simulink subsystem "Shooting_Parameters_sub"  (R2023b)
settings: Solver=VariableStepAuto  StartTime=0.0  StopTime=10.0  RelTol=1e-3
undefined symbols (not defined in the file): Blue_Hub_LeftX, Blue_Hub_LeftY, Blue_Hub_RightX, Blue_Hub_RightY, Field_Blue_Hub_X, Field_Blue_Pass_X, Field_Hub_Y, Field_Length, Field_Length_Half, Field_Pass_Y_Bottom, Field_Pass_Y_Top, Field_Red_Hub_X, Field_Red_Pass_X, Field_Width_Pass, iterations, Rebuilt_Des_Gyro_Shoot_Offset, Rebuilt_Shoot_Dist_0, Rebuilt_Shoot_Dist_1, Rebuilt_Shoot_Dist_2, Rebuilt_Shoot_Dist_3, Rebuilt_Shoot_Dist_4, Rebuilt_Shoot_Dist_5, Rebuilt_Shoot_Dist_6, Rebuilt_Shoot_Dist_7, Rebuilt_Shoot_Gyro_Err_0, Rebuilt_Shoot_Gyro_Err_1, Rebuilt_Shoot_Gyro_Err_2, Rebuilt_Shoot_Gyro_Err_3, Rebuilt_Shoot_Gyro_Err_4, Rebuilt_Shoot_Gyro_Err_5, Rebuilt_Shoot_Gyro_Err_6, Rebuilt_Shoot_Gyro_Err_7, Rebuilt_Shoot_Hood_Pos_0, Rebuilt_Shoot_Hood_Pos_1, Rebuilt_Shoot_Hood_Pos_2, Rebuilt_Shoot_Hood_Pos_3, Rebuilt_Shoot_Hood_Pos_4, Rebuilt_Shoot_Hood_Pos_5, Rebuilt_Shoot_Hood_Pos_6, Rebuilt_Shoot_Hood_Pos_7, Rebuilt_Shoot_Shooter_Spd_0, Rebuilt_Shoot_Shooter_Spd_1, Rebuilt_Shoot_Shooter_Spd_2, Rebuilt_Shoot_Shooter_Spd_3, Rebuilt_Shoot_Shooter_Spd_4, Rebuilt_Shoot_Shooter_Spd_5, Rebuilt_Shoot_Shooter_Spd_6, Rebuilt_Shoot_Shooter_Spd_7, Rebuilt_Shoot_Shooter_Spd_I_0, Rebuilt_Shoot_Shooter_Spd_I_1, Rebuilt_Shoot_Shooter_Spd_I_2, Rebuilt_Shoot_Shooter_Spd_I_3, Rebuilt_Shoot_Shooter_Spd_I_4, Rebuilt_Shoot_Shooter_Spd_I_5, Rebuilt_Shoot_Shooter_Spd_I_6, Rebuilt_Shoot_Shooter_Spd_I_7, Rebuilt_Shoot_Target_Error_Thresh, Rebuilt_Shoot_TOF_0, Rebuilt_Shoot_TOF_1, Rebuilt_Shoot_TOF_2 ... (+11)
libraries: simulink x6, simulink_extras x2
settings Model: Creator=ander  LastModifiedBy=FIRSTMentor

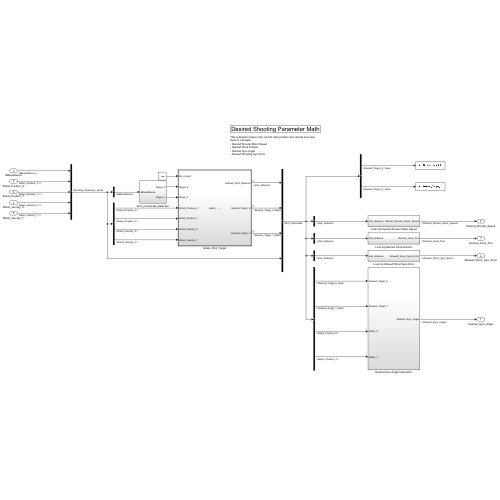
[thumbnail: Simulink's stored preview of the top-level diagram]
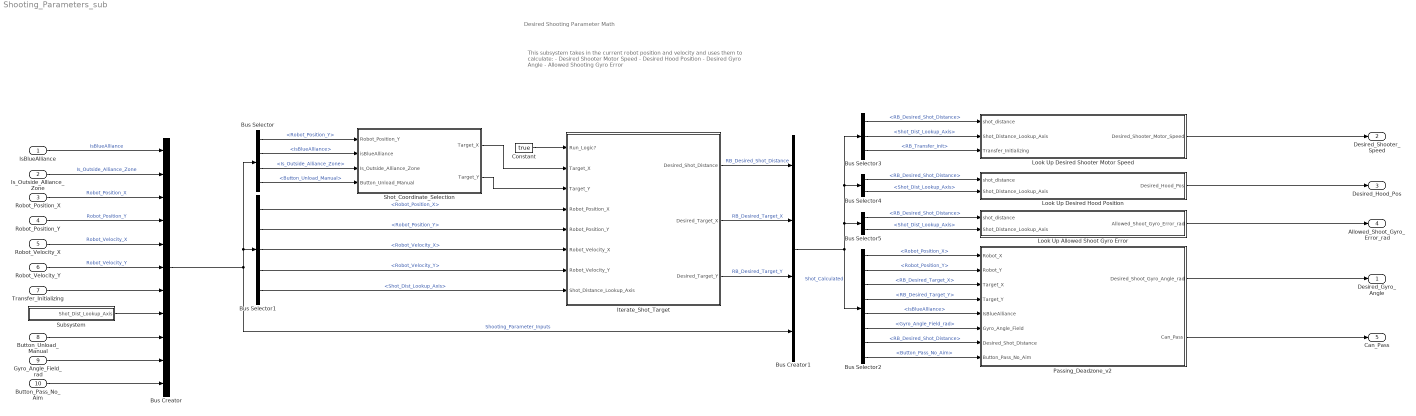
== system Shooting_Parameters_sub ==
  note: Desired Shooting Parameter Math
  note: This subsystem takes in the current robot position and velocity and uses them to calculate:
      | - Desired Shooter Motor Speed
      | - Desired Hood Position
      | - Desired Gyro Angle
      | - Allowed Shooting Gyro Error
  IsBlueAlliance : Inport
  Is_Outside_Alliance_Zone : Inport  Port=2
  Robot_Position_X : Inport  Port=3
  Robot_Position_Y : Inport  Port=4
  Robot_Velocity_X : Inport  Port=5
  Robot_Velocity_Y : Inport  Port=6
  Transfer_Initializing : Inport  Port=7
  Button_Unload_Manual : Inport  Port=8
  Gyro_Angle_Field_rad : Inport  Port=9
  Button_Pass_No_Aim : Inport  Port=10
  Bus Creator : BusCreator  Inputs=11
  Bus Creator1 : BusCreator  Inputs=4
  Bus Selector : BusSelector  OutputSignals=Robot_Position_Y,IsBlueAlliance,Is_Outside_Alliance_Zone,Button_Unload_Manual
  Bus Selector1 : BusSelector  OutputSignals=Robot_Position_X,Robot_Position_Y,Robot_Velocity_X,Robot_Velocity_Y,Shot_Dist_Lookup_Axis
  Bus Selector2 : BusSelector  OutputSignals=Shooting_Parameter_Inputs.Robot_Position_X,Shooting_Parameter_Inputs.Robot_Position_Y,RB_Desired_Target_X,RB_Desired_Target_Y,Shooting_Parameter_Inputs.IsBlueAlliance,Shooting_Parameter_Inputs.Gyro_Angle_Field_rad,RB_Desired_Shot_Distance,Shooting_Parameter_Inputs.Button_Pass_No_Aim
  Bus Selector3 : BusSelector  OutputSignals=RB_Desired_Shot_Distance,Shooting_Parameter_Inputs.Shot_Dist_Lookup_Axis,Shooting_Parameter_Inputs.RB_Transfer_Init
  Bus Selector4 : BusSelector  OutputSignals=RB_Desired_Shot_Distance,Shooting_Parameter_Inputs.Shot_Dist_Lookup_Axis
  Bus Selector5 : BusSelector  OutputSignals=RB_Desired_Shot_Distance,Shooting_Parameter_Inputs.Shot_Dist_Lookup_Axis
  Constant : Constant  Value=true  OutDataTypeStr=boolean
  Iterate_Shot_Target : Subsystem  TreatAsAtomicUnit=on
  Look Up Allowed Shoot Gyro Error : Subsystem
  Look Up Desired Hood Position : Subsystem
  Look Up Desired Shooter Motor Speed : Subsystem
  Passing_Deadzone_v2 : Subsystem
  Shot_Coordinate_Selection : Subsystem
  Subsystem : Subsystem
  Desired_Gyro_Angle : Outport
  Desired_Shooter_Speed : Outport  Port=2
  Desired_Hood_Pos : Outport  Port=3
  Allowed_Shoot_Gyro_Error_rad : Outport  Port=4
  Can_Pass : Outport  Port=5
  wires:
  Robot_Position_X/1 -> Bus Creator/3  "Robot_Position_X"
  Constant/1 -> Iterate_Shot_Target/1(Run_Logic?)
  Bus Selector1/2 -> Iterate_Shot_Target/5(Robot_Position_Y)  "<Robot_Position_Y>"
  Look Up Desired Hood Position/1(Desired_Hood_Pos) -> Desired_Hood_Pos/1
  Robot_Position_Y/1 -> Bus Creator/4  "Robot_Position_Y"
  Bus Selector/2 -> Shot_Coordinate_Selection/2(isBlueAlliance)  "<IsBlueAlliance>"
  Iterate_Shot_Target/2(Desired_Target_X) -> Bus Creator1/2  "RB_Desired_Target_X"
  Bus Selector4/1 -> Look Up Desired Hood Position/1(shot_distance)  "<RB_Desired_Shot_Distance>"
  Shot_Coordinate_Selection/1(Target_X) -> Iterate_Shot_Target/2(Target_X)
  Bus Creator/1 -> Bus Creator1/4, Bus Selector1/1, Bus Selector/1  "Shooting_Parameter_Inputs"
  Look Up Desired Shooter Motor Speed/1(Desired_Shooter_Motor_Speed) -> Desired_Shooter_Speed/1
  Bus Creator1/1 -> Bus Selector2/1, Bus Selector5/1, Bus Selector3/1, Bus Selector4/1  "Shot_Calculated"
  Shot_Coordinate_Selection/2(Target_Y) -> Iterate_Shot_Target/3(Target_Y)
  Bus Selector3/1 -> Look Up Desired Shooter Motor Speed/1(shot_distance)  "<RB_Desired_Shot_Distance>"
  Robot_Velocity_X/1 -> Bus Creator/5  "Robot_Velocity_X"
  Bus Selector5/1 -> Look Up Allowed Shoot Gyro Error/1(shot_distance)  "<RB_Desired_Shot_Distance>"
  Iterate_Shot_Target/1(Desired_Shot_Distance) -> Bus Creator1/1  "RB_Desired_Shot_Distance"
  Bus Selector1/4 -> Iterate_Shot_Target/7(Robot_Velocity_Y)  "<Robot_Velocity_Y>"
  Bus Selector1/1 -> Iterate_Shot_Target/4(Robot_Position_X)  "<Robot_Position_X>"
  Bus Selector1/3 -> Iterate_Shot_Target/6(Robot_Velocity_X)  "<Robot_Velocity_X>"
  Robot_Velocity_Y/1 -> Bus Creator/6  "Robot_Velocity_Y"
  Look Up Allowed Shoot Gyro Error/1(Allowed_Shoot_Gyro_Error_rad) -> Allowed_Shoot_Gyro_Error_rad/1
  Iterate_Shot_Target/3(Desired_Target_Y) -> Bus Creator1/3  "RB_Desired_Target_Y"
  Subsystem/1(Shot_Dist_Lookup_Axis) -> Bus Creator/8
  Bus Selector3/2 -> Look Up Desired Shooter Motor Speed/2(Shot_Distance_Lookup_Axis)  "<Shot_Dist_Lookup_Axis>"
  Bus Selector5/2 -> Look Up Allowed Shoot Gyro Error/2(Shot_Distance_Lookup_Axis)  "<Shot_Dist_Lookup_Axis>"
  Bus Selector4/2 -> Look Up Desired Hood Position/2(Shot_Distance_Lookup_Axis)  "<Shot_Dist_Lookup_Axis>"
  Bus Selector1/5 -> Iterate_Shot_Target/8(Shot_Distance_Lookup_Axis)  "<Shot_Dist_Lookup_Axis>"
  Bus Selector/1 -> Shot_Coordinate_Selection/1(Robot_Position_Y)  "<Robot_Position_Y>"
  Bus Selector/3 -> Shot_Coordinate_Selection/3(Is_Outside_Alliance_Zone)  "<Is_Outside_Alliance_Zone>"
  IsBlueAlliance/1 -> Bus Creator/1  "IsBlueAlliance"
  Is_Outside_Alliance_Zone/1 -> Bus Creator/2  "Is_Outside_Alliance_Zone"
  Transfer_Initializing/1 -> Bus Creator/7
  Bus Selector3/3 -> Look Up Desired Shooter Motor Speed/3(Transfer_Initializing)  "<RB_Transfer_Init>"
  Button_Unload_Manual/1 -> Bus Creator/9
  Bus Selector/4 -> Shot_Coordinate_Selection/4(Button_Unload_Manual)  "<Button_Unload_Manual>"
  Gyro_Angle_Field_rad/1 -> Bus Creator/10
  Button_Pass_No_Aim/1 -> Bus Creator/11
  Bus Selector2/1 -> Passing_Deadzone_v2/1(Robot_X)  "<Robot_Position_X>"
  Bus Selector2/2 -> Passing_Deadzone_v2/2(Robot_Y)  "<Robot_Position_Y>"
  Bus Selector2/3 -> Passing_Deadzone_v2/3(Target_X)  "<RB_Desired_Target_X>"
  Bus Selector2/4 -> Passing_Deadzone_v2/4(Target_Y)  "<RB_Desired_Target_Y>"
  Bus Selector2/5 -> Passing_Deadzone_v2/5(IsBlueAlliance)  "<IsBlueAlliance>"
  Bus Selector2/6 -> Passing_Deadzone_v2/6(Gyro_Angle_Field)  "<Gyro_Angle_Field_rad>"
  Bus Selector2/7 -> Passing_Deadzone_v2/7(Desired_Shot_Distance)  "<RB_Desired_Shot_Distance>"
  Bus Selector2/8 -> Passing_Deadzone_v2/8(Button_Pass_No_Aim)  "<Button_Pass_No_Aim>"
  Passing_Deadzone_v2/1(Desired_Shoot_Gyro_Angle_rad) -> Desired_Gyro_Angle/1
  Passing_Deadzone_v2/2(Can_Pass) -> Can_Pass/1

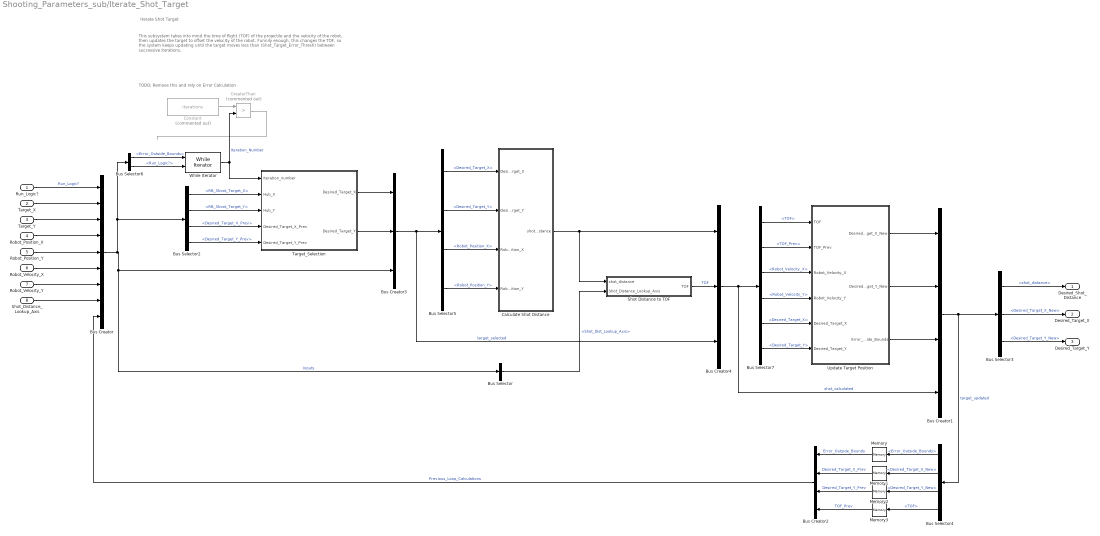
== system Shooting_Parameters_sub/Iterate_Shot_Target ==
  note: Iterate Shot Target
  note: This subsystem takes into mind the time of flight (TOF) of the projectile and the velocity of the robot, then updates the target to offset the velocity of the robot. Funnily enough, this changes the TOF, so the system keeps updating until the target moves less than (Shot_Target_Error_Thresh) between successive iterations.
  note: TODO: Remove this and rely on Error Calculation
  Run_Logic? : Inport
  Target_X : Inport  Port=2
  Target_Y : Inport  Port=3
  Robot_Position_X : Inport  Port=4
  Robot_Position_Y : Inport  Port=5
  Robot_Velocity_X : Inport  Port=6
  Robot_Velocity_Y : Inport  Port=7
  Shot_Distance_Lookup_Axis : Inport  Port=8
  Bus Creator : BusCreator  Inputs=9
  Bus Creator1 : BusCreator  Inputs=4
  Bus Creator2 : BusCreator  Inputs=4
  Bus Creator3 : BusCreator  Inputs=3
  Bus Creator4 : BusCreator  Inputs=3
  Bus Selector : BusSelector  OutputSignals=Shot_Dist_Lookup_Axis
  Bus Selector2 : BusSelector  OutputSignals=RB_Shoot_Target_X,RB_Shoot_Target_Y,Previous_Loop_Calculations.Desired_Target_X_Prev,Previous_Loop_Calculations.Desired_Target_Y_Prev
  Bus Selector3 : BusSelector  OutputSignals=shot_calculated.shot_distance,Desired_Target_X_New,Desired_Target_Y_New
  Bus Selector4 : BusSelector  OutputSignals=Error_Outside_Bounds,Desired_Target_X_New,Desired_Target_Y_New,shot_calculated.TOF
  Bus Selector5 : BusSelector  OutputSignals=Desired_Target_X,Desired_Target_Y,Inputs.Robot_Position_X,Inputs.Robot_Position_Y
  Bus Selector6 : BusSelector  OutputSignals=Previous_Loop_Calculations.Error_Outside_Bounds,Run_Logic?
  Bus Selector7 : BusSelector  OutputSignals=TOF,target_selected.Inputs.Previous_Loop_Calculations.TOF_Prev,target_selected.Inputs.Robot_Velocity_X,target_selected.Inputs.Robot_Velocity_Y,target_selected.Desired_Target_X,target_selected.Desired_Target_Y
  Calculate Shot Distance : Subsystem
  Constant : Constant  Commented=on  Value=iterations
  GreaterThan : RelationalOperator  Commented=on  Operator=>  OutDataTypeStr=boolean  RndMeth=Simplest  InputSameDT=off
  Memory : Memory  InitialCondition=true  InheritSampleTime=on
  Memory1 : Memory  InheritSampleTime=on
  Memory2 : Memory  InheritSampleTime=on
  Memory3 : Memory  InheritSampleTime=on
  Shot Distance to TOF : Subsystem
  Target_Selection : Subsystem
  Update Target Position : Subsystem
  While Iterator : WhileIterator  MaxIters=10  ResetStates=reset  ShowIterationPort=on  OutputDataType=uint8
  Desired_Shot_Distance : Outport
  Desired_Target_X : Outport  Port=2
  Desired_Target_Y : Outport  Port=3
  wires:
  Bus Selector/1 -> Shot Distance to TOF/2(Shot_Distance_Lookup_Axis)  "<Shot_Dist_Lookup_Axis>"
  Shot_Distance_Lookup_Axis/1 -> Bus Creator/8
  Robot_Velocity_Y/1 -> Bus Creator/7
  Robot_Velocity_X/1 -> Bus Creator/6
  Robot_Position_Y/1 -> Bus Creator/5
  GreaterThan/1 -> ?
  Constant/1 -> GreaterThan/1
  Bus Selector7/2 -> Update Target Position/2(TOF_Prev)  "<TOF_Prev>"
  Bus Selector3/1 -> Desired_Shot_Distance/1  "<shot_distance>"
  Bus Selector7/6 -> Update Target Position/6(Desired_Target_Y)  "<Desired_Target_Y>"
  Bus Selector7/5 -> Update Target Position/5(Desired_Target_X)  "<Desired_Target_X>"
  Bus Selector7/4 -> Update Target Position/4(Robot_Velocity_Y)  "<Robot_Velocity_Y>"
  Bus Selector7/3 -> Update Target Position/3(Robot_Velocity_X)  "<Robot_Velocity_X>"
  Bus Selector7/1 -> Update Target Position/1(TOF)  "<TOF>"
  Bus Creator4/1 -> Bus Creator1/4, Bus Selector7/1  "shot_calculated"
  Bus Selector4/4 -> Memory3/1  "<TOF>"
  Memory3/1 -> Bus Creator2/4  "TOF_Prev"
  Bus Selector5/4 -> Calculate Shot Distance/4(Robot_Position_Y)  "<Robot_Position_Y>"
  Bus Selector5/3 -> Calculate Shot Distance/3(Robot_Position_X)  "<Robot_Position_X>"
  Bus Selector5/2 -> Calculate Shot Distance/2(Desired_Target_Y)  "<Desired_Target_Y>"
  Bus Selector5/1 -> Calculate Shot Distance/1(Desired_Target_X)  "<Desired_Target_X>"
  Bus Creator3/1 -> Bus Selector5/1, Bus Creator4/3  "target_selected"
  Target_Selection/2(Desired_Target_Y) -> Bus Creator3/2
  Target_Selection/1(Desired_Target_X) -> Bus Creator3/1
  Bus Selector2/4 -> Target_Selection/5(Desired_Target_Y_Prev)  "<Desired_Target_Y_Prev>"
  Bus Selector2/3 -> Target_Selection/4(Desired_Target_X_Prev)  "<Desired_Target_X_Prev>"
  Bus Selector6/2 -> While Iterator/2  "<Run_Logic?>"
  Bus Selector6/1 -> While Iterator/1  "<Error_Outside_Bounds>"
  Bus Creator2/1 -> Bus Creator/9  "Previous_Loop_Calculations"
  Memory/1 -> Bus Creator2/1  "Error_Outside_Bounds"
  Memory2/1 -> Bus Creator2/3  "Desired_Target_Y_Prev"
  Memory1/1 -> Bus Creator2/2  "Desired_Target_X_Prev"
  Bus Selector4/3 -> Memory2/1  "<Desired_Target_Y_New>"
  Bus Selector4/2 -> Memory1/1  "<Desired_Target_X_New>"
  Bus Selector4/1 -> Memory/1  "<Error_Outside_Bounds>"
  Update Target Position/3(Error_Outside_Bounds) -> Bus Creator1/3
  Bus Selector3/3 -> Desired_Target_Y/1  "<Desired_Target_Y_New>"
  Bus Creator1/1 -> Bus Selector4/1, Bus Selector3/1  "target_updated"
  Bus Selector3/2 -> Desired_Target_X/1  "<Desired_Target_X_New>"
  Bus Selector2/2 -> Target_Selection/3(Hub_Y)  "<RB_Shoot_Target_Y>"
  Bus Selector2/1 -> Target_Selection/2(Hub_X)  "<RB_Shoot_Target_X>"
  Update Target Position/2(Desired_Target_Y_New) -> Bus Creator1/2
  Update Target Position/1(Desired_Target_X_New) -> Bus Creator1/1
  Bus Creator/1 -> Bus Selector2/1, Bus Selector6/1, Bus Creator3/3, Bus Selector/1  "Inputs"
  Target_X/1 -> Bus Creator/2
  Robot_Position_X/1 -> Bus Creator/4
  Target_Y/1 -> Bus Creator/3
  Shot Distance to TOF/1(TOF) -> Bus Creator4/2  "TOF"
  Calculate Shot Distance/1(shot_distance) -> Bus Creator4/1, Shot Distance to TOF/1(shot_distance)
  While Iterator/1 -> Target_Selection/1(iteration_number), GreaterThan/2  "Iteration_Number"
  Run_Logic?/1 -> Bus Creator/1  "Run_Logic?"

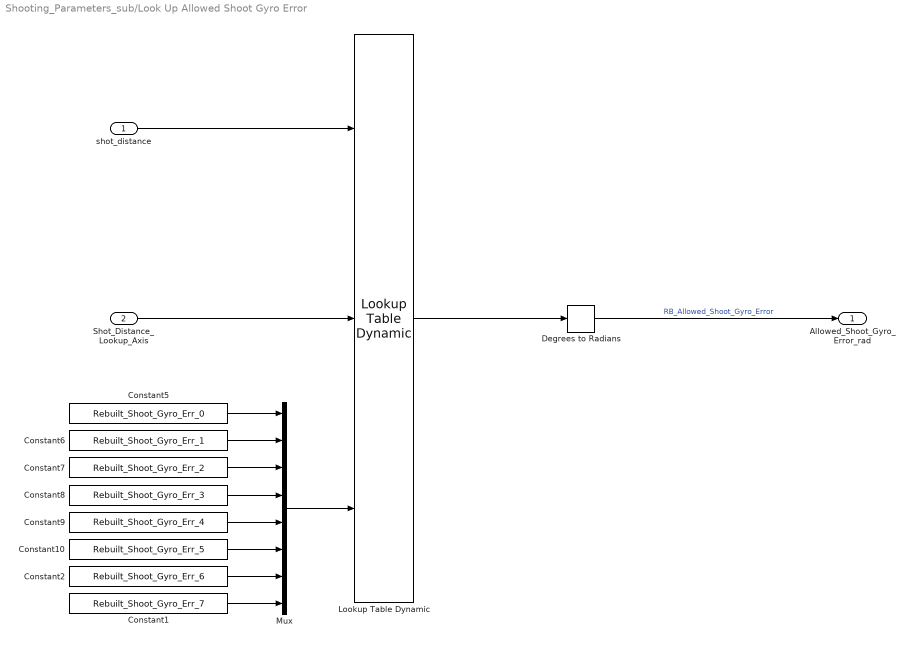
== system Shooting_Parameters_sub/Look Up Allowed Shoot Gyro Error ==
  shot_distance : Inport
  Shot_Distance_Lookup_Axis : Inport  Port=2
  Constant1 : Constant  Value=Rebuilt_Shoot_Gyro_Err_7
  Constant10 : Constant  Value=Rebuilt_Shoot_Gyro_Err_5
  Constant2 : Constant  Value=Rebuilt_Shoot_Gyro_Err_6
  Constant5 : Constant  Value=Rebuilt_Shoot_Gyro_Err_0
  Constant6 : Constant  Value=Rebuilt_Shoot_Gyro_Err_1
  Constant7 : Constant  Value=Rebuilt_Shoot_Gyro_Err_2
  Constant8 : Constant  Value=Rebuilt_Shoot_Gyro_Err_3
  Constant9 : Constant  Value=Rebuilt_Shoot_Gyro_Err_4
  Degrees to Radians : simulink_extras/Transformations/Degrees to Radians
  Lookup Table Dynamic : simulink/Lookup Tables/Lookup Table Dynamic  LookUpMeth=Interpolation-Use End Values  OutDataType=fixdt('double')  OutScaling=[]  OutputDataTypeScalingMode=Specify via dialog  OutDataTypeStr=double  DoSatur=off
  Mux : Mux  Inputs=8
  Allowed_Shoot_Gyro_Error_rad : Outport
  wires:
  Constant6/1 -> Mux/2
  Constant10/1 -> Mux/6
  Constant9/1 -> Mux/5
  Constant1/1 -> Mux/8
  Constant5/1 -> Mux/1
  Constant2/1 -> Mux/7
  Constant7/1 -> Mux/3
  Constant8/1 -> Mux/4
  Mux/1 -> Lookup Table Dynamic/3
  Shot_Distance_Lookup_Axis/1 -> Lookup Table Dynamic/2
  Degrees to Radians/1 -> Allowed_Shoot_Gyro_Error_rad/1  "RB_Allowed_Shoot_Gyro_Error"
  Lookup Table Dynamic/1 -> Degrees to Radians/1
  shot_distance/1 -> Lookup Table Dynamic/1

== system Shooting_Parameters_sub/Look Up Desired Hood Position ==
  shot_distance : Inport
  Shot_Distance_Lookup_Axis : Inport  Port=2
  Constant1 : Constant  Value=Rebuilt_Shoot_Hood_Pos_7
  Constant10 : Constant  Value=Rebuilt_Shoot_Hood_Pos_5
  Constant2 : Constant  Value=Rebuilt_Shoot_Hood_Pos_6
  Constant5 : Constant  Value=Rebuilt_Shoot_Hood_Pos_0
  Constant6 : Constant  Value=Rebuilt_Shoot_Hood_Pos_1
  Constant7 : Constant  Value=Rebuilt_Shoot_Hood_Pos_2
  Constant8 : Constant  Value=Rebuilt_Shoot_Hood_Pos_3
  Constant9 : Constant  Value=Rebuilt_Shoot_Hood_Pos_4
  Lookup Table Dynamic : simulink/Lookup Tables/Lookup Table Dynamic  LookUpMeth=Interpolation-Use End Values  OutDataType=fixdt('double')  OutScaling=[]  OutputDataTypeScalingMode=Specify via dialog  OutDataTypeStr=double  DoSatur=off
  Mux : Mux  Inputs=8
  Desired_Hood_Pos : Outport
  wires:
  Mux/1 -> Lookup Table Dynamic/3
  Constant2/1 -> Mux/7
  Constant6/1 -> Mux/2
  Constant10/1 -> Mux/6
  Constant1/1 -> Mux/8
  Constant5/1 -> Mux/1
  Constant9/1 -> Mux/5
  Constant7/1 -> Mux/3
  Constant8/1 -> Mux/4
  Shot_Distance_Lookup_Axis/1 -> Lookup Table Dynamic/2
  Lookup Table Dynamic/1 -> Desired_Hood_Pos/1
  shot_distance/1 -> Lookup Table Dynamic/1

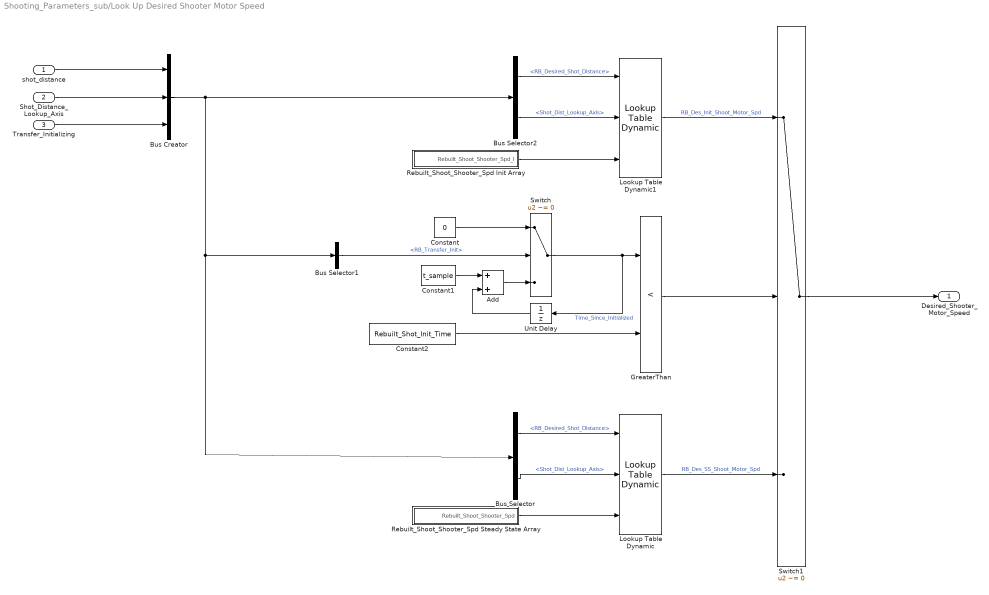
== system Shooting_Parameters_sub/Look Up Desired Shooter Motor Speed ==
  shot_distance : Inport
  Shot_Distance_Lookup_Axis : Inport  Port=2
  Transfer_Initializing : Inport  Port=3
  Add : Sum
  Bus Creator : BusCreator  Inputs=3
  Bus Selector : BusSelector  OutputSignals=RB_Desired_Shot_Distance,Shot_Dist_Lookup_Axis
  Bus Selector1 : BusSelector  OutputSignals=RB_Transfer_Init
  Bus Selector2 : BusSelector  OutputSignals=RB_Desired_Shot_Distance,Shot_Dist_Lookup_Axis
  Constant : Constant  Value=0
  Constant1 : Constant  Value=t_sample
  Constant2 : Constant  Value=Rebuilt_Shot_Init_Time
  GreaterThan : RelationalOperator  Operator=<  OutDataTypeStr=boolean  RndMeth=Simplest  InputSameDT=off
  Lookup Table Dynamic : simulink/Lookup Tables/Lookup Table Dynamic  LookUpMeth=Interpolation-Use End Values  OutDataType=fixdt('double')  OutScaling=[]  OutputDataTypeScalingMode=Specify via dialog  OutDataTypeStr=double  DoSatur=off
  Lookup Table Dynamic1 : simulink/Lookup Tables/Lookup Table Dynamic  LookUpMeth=Interpolation-Use End Values  OutDataType=fixdt('double')  OutScaling=[]  OutputDataTypeScalingMode=Specify via dialog  OutDataTypeStr=double  DoSatur=off
  Rebuilt_Shoot_Shooter_Spd Init Array : Subsystem
  Rebuilt_Shoot_Shooter_Spd Steady State Array : Subsystem
  Switch : Switch  Criteria=u2 ~= 0  SaturateOnIntegerOverflow=off  InputSameDT=off
  Switch1 : Switch  Criteria=u2 ~= 0  SaturateOnIntegerOverflow=off  InputSameDT=off
  Unit Delay : UnitDelay  SampleTime=-1  HasFrameUpgradeWarning=on
  Desired_Shooter_Motor_Speed : Outport
  wires:
  GreaterThan/1 -> Switch1/2
  Lookup Table Dynamic/1 -> Switch1/3  "RB_Des_SS_Shoot_Motor_Spd"
  Lookup Table Dynamic1/1 -> Switch1/1  "RB_Des_Init_Shoot_Motor_Spd"
  Rebuilt_Shoot_Shooter_Spd Init Array/1(Rebuilt_Shoot_Shooter_Spd_I) -> Lookup Table Dynamic1/3
  Bus Selector2/1 -> Lookup Table Dynamic1/1  "<RB_Desired_Shot_Distance>"
  Bus Selector2/2 -> Lookup Table Dynamic1/2  "<Shot_Dist_Lookup_Axis>"
  Bus Creator/1 -> Bus Selector1/1, Bus Selector/1, Bus Selector2/1
  Constant2/1 -> GreaterThan/2
  Add/1 -> Switch/3
  Constant1/1 -> Add/1
  Unit Delay/1 -> Add/2
  Constant/1 -> Switch/1
  Switch/1 -> GreaterThan/1, Unit Delay/1  "Time_Since_Initialized"
  Bus Selector1/1 -> Switch/2  "<RB_Transfer_Init>"
  Rebuilt_Shoot_Shooter_Spd Steady State Array/1(Rebuilt_Shoot_Shooter_Spd) -> Lookup Table Dynamic/3
  Bus Selector/2 -> Lookup Table Dynamic/2  "<Shot_Dist_Lookup_Axis>"
  Bus Selector/1 -> Lookup Table Dynamic/1  "<RB_Desired_Shot_Distance>"
  Transfer_Initializing/1 -> Bus Creator/3
  Shot_Distance_Lookup_Axis/1 -> Bus Creator/2
  Switch1/1 -> Desired_Shooter_Motor_Speed/1
  shot_distance/1 -> Bus Creator/1

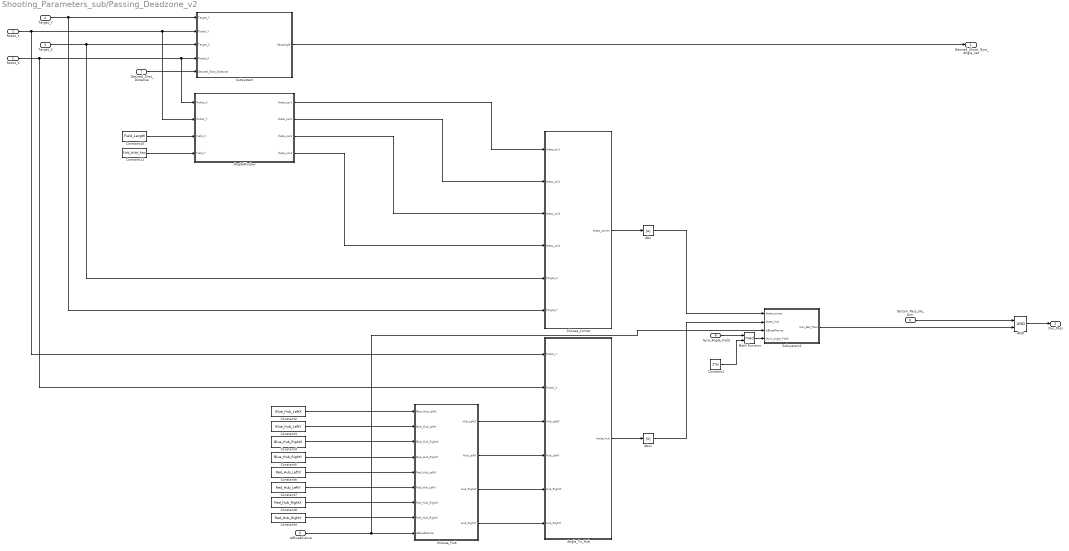
== system Shooting_Parameters_sub/Passing_Deadzone_v2 ==
  Robot_X : Inport
  Robot_Y : Inport  Port=2
  Target_X : Inport  Port=3
  Target_Y : Inport  Port=4
  IsBlueAlliance : Inport  Port=5
  Gyro_Angle_Field : Inport  Port=6
  Desired_Shot_Distance : Inport  Port=7
  Button_Pass_No_Aim : Inport  Port=8
  AND : Logic  AllPortsSameDT=off  OutDataTypeStr=boolean
  Abs : Abs  SaturateOnIntegerOverflow=off
  Abs1 : Abs  SaturateOnIntegerOverflow=off
  AngleWindow : Subsystem
  Angle_To_Hub : Subsystem
  Choose_Corner : Subsystem
  Choose_Hub : Subsystem
  Constant1 : Constant  Value=2*pi
  Constant10 : Constant  Value=Field_Length
  Constant11 : Constant  Value=Field_Width_Pass
  Constant2 : Constant  Value=Blue_Hub_LeftX
  Constant3 : Constant  Value=Blue_Hub_LeftY
  Constant4 : Constant  Value=Blue_Hub_RightX
  Constant5 : Constant  Value=Blue_Hub_RightY
  Constant6 : Constant  Value=Red_Hub_LeftX
  Constant7 : Constant  Value=Red_Hub_LeftY
  Constant8 : Constant  Value=Red_Hub_RightX
  Constant9 : Constant  Value=Red_Hub_RightY
  Math Function : Math  Operator=mod
  Subsystem : Subsystem
  Subsystem1 : Subsystem
  Desired_Shoot_Gyro_Angle_rad : Outport
  Can_Pass : Outport  Port=2
  wires:
  Button_Pass_No_Aim/1 -> AND/1
  Math Function/1 -> Subsystem1/4(Gyro_Angle_Field)
  Gyro_Angle_Field/1 -> Math Function/1
  Constant1/1 -> Math Function/2
  Subsystem1/1(Can_Bot_Pass) -> AND/2
  Abs1/1 -> Subsystem1/2(theta_hub)
  Abs/1 -> Subsystem1/1(theta_corner)
  AND/1 -> Can_Pass/1
  Desired_Shot_Distance/1 -> Subsystem/5(Desired_Shot_Distance)
  Constant11/1 -> AngleWindow/4(Field_Y)
  Constant3/1 -> Choose_Hub/2(Blue_Hub_LeftY)
  Subsystem/1(PassAngle) -> Desired_Shoot_Gyro_Angle_rad/1
  Angle_To_Hub/1(theta_hub) -> Abs1/1
  Choose_Corner/1(theta_corner) -> Abs/1
  Choose_Hub/4(Hub_RightY) -> Angle_To_Hub/6(Hub_RightY)
  Choose_Hub/3(Hub_RightX) -> Angle_To_Hub/5(Hub_RightX)
  Choose_Hub/2(Hub_LeftY) -> Angle_To_Hub/4(Hub_LeftY)
  Choose_Hub/1(Hub_LeftX) -> Angle_To_Hub/3(Hub_LeftX)
  IsBlueAlliance/1 -> Choose_Hub/9(IsBlueAlliance), Subsystem1/3(IsBlueAlliance)
  Constant9/1 -> Choose_Hub/8(Red_Hub_RightY)
  Constant8/1 -> Choose_Hub/7(Red_Hub_RightX)
  Constant7/1 -> Choose_Hub/6(Red_Hub_LeftY)
  Constant6/1 -> Choose_Hub/5(Red_Hub_LeftX)
  Constant5/1 -> Choose_Hub/4(Blue_Hub_RightY)
  Constant4/1 -> Choose_Hub/3(Blue_Hub_RightX)
  Constant2/1 -> Choose_Hub/1(Blue_Hub_LeftX)
  AngleWindow/4(theta_cor4) -> Choose_Corner/4(theta_cor4)
  AngleWindow/3(theta_cor3) -> Choose_Corner/3(theta_cor3)
  AngleWindow/2(theta_cor2) -> Choose_Corner/2(theta_cor2)
  AngleWindow/1(theta_cor1) -> Choose_Corner/1(theta_cor1)
  Constant10/1 -> AngleWindow/3(Field_X)
  Robot_X/1 -> Angle_To_Hub/2(Robot_X), Subsystem/4(Robot_X), AngleWindow/1(Robot_X)
  Target_X/1 -> Subsystem/3(Target_X), Choose_Corner/5(Target_X)
  Robot_Y/1 -> Subsystem/2(Robot_Y), AngleWindow/2(Robot_Y), Angle_To_Hub/1(Robot_Y)
  Target_Y/1 -> Subsystem/1(Target_Y), Choose_Corner/6(Target_Y)

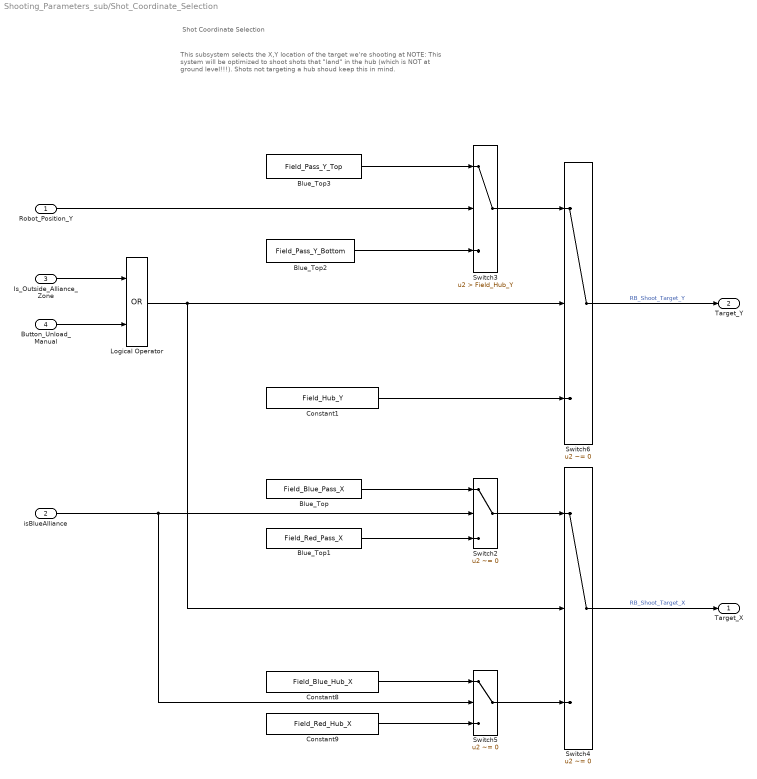
== system Shooting_Parameters_sub/Shot_Coordinate_Selection ==
  note: Shot Coordinate Selection
  note: This subsystem selects the X,Y location of the target we're shooting at
      |
      | NOTE: This system will be optimized to shoot shots that "land" in the hub (which is NOT at ground level!!!). Shots not targeting a hub shoud keep this in mind.
  Robot_Position_Y : Inport
  isBlueAlliance : Inport  Port=2
  Is_Outside_Alliance_Zone : Inport  Port=3
  Button_Unload_Manual : Inport  Port=4
  Blue_Top : Constant  Value=Field_Blue_Pass_X
  Blue_Top1 : Constant  Value=Field_Red_Pass_X
  Blue_Top2 : Constant  Value=Field_Pass_Y_Bottom
  Blue_Top3 : Constant  Value=Field_Pass_Y_Top
  Constant1 : Constant  Value=Field_Hub_Y
  Constant8 : Constant  Value=Field_Blue_Hub_X
  Constant9 : Constant  Value=Field_Red_Hub_X
  Logical Operator : Logic  Operator=OR  AllPortsSameDT=off  OutDataTypeStr=boolean
  Switch{2,4..6} (4 alike) : Switch  Criteria=u2 ~= 0  SaturateOnIntegerOverflow=off  InputSameDT=off
  Switch3 : Switch  Criteria=u2 > Threshold  Threshold=Field_Hub_Y  SaturateOnIntegerOverflow=off  InputSameDT=off
      settings: AttributesFormatString=Threshold = %<Threshold>
  Target_X : Outport
  Target_Y : Outport  Port=2
  wires:
  Button_Unload_Manual/1 -> Logical Operator/2
  Is_Outside_Alliance_Zone/1 -> Logical Operator/1
  Constant1/1 -> Switch6/3
  Blue_Top1/1 -> Switch2/3
  Blue_Top/1 -> Switch2/1
  Switch2/1 -> Switch4/1
  Switch5/1 -> Switch4/3
  Blue_Top2/1 -> Switch3/3
  Blue_Top3/1 -> Switch3/1
  Switch3/1 -> Switch6/1
  Switch6/1 -> Target_Y/1  "RB_Shoot_Target_Y"
  Switch4/1 -> Target_X/1  "RB_Shoot_Target_X"
  Constant9/1 -> Switch5/3
  Constant8/1 -> Switch5/1
  isBlueAlliance/1 -> Switch2/2, Switch5/2
  Logical Operator/1 -> Switch6/2, Switch4/2
  Robot_Position_Y/1 -> Switch3/2

== system Shooting_Parameters_sub/Subsystem ==
  Constant1 : Constant  Value=Rebuilt_Shoot_Dist_7
  Constant10 : Constant  Value=Rebuilt_Shoot_Dist_5
  Constant2 : Constant  Value=Rebuilt_Shoot_Dist_6
  Constant5 : Constant  Value=Rebuilt_Shoot_Dist_0
  Constant6 : Constant  Value=Rebuilt_Shoot_Dist_1
  Constant7 : Constant  Value=Rebuilt_Shoot_Dist_2
  Constant8 : Constant  Value=Rebuilt_Shoot_Dist_3
  Constant9 : Constant  Value=Rebuilt_Shoot_Dist_4
  Mux : Mux  Inputs=8
  Shot_Dist_Lookup_Axis : Outport
  wires:
  Mux/1 -> Shot_Dist_Lookup_Axis/1  "Shot_Dist_Lookup_Axis"
  Constant5/1 -> Mux/1
  Constant6/1 -> Mux/2
  Constant10/1 -> Mux/6
  Constant1/1 -> Mux/8
  Constant9/1 -> Mux/5
  Constant8/1 -> Mux/4
  Constant7/1 -> Mux/3
  Constant2/1 -> Mux/7

== system Shooting_Parameters_sub/Iterate_Shot_Target/Calculate Shot Distance ==
  note: Calculate Shot Distance
  note: This subsystem takes a simple distance between 2 points.
  Desired_Target_X : Inport
  Desired_Target_Y : Inport  Port=2
  Robot_Position_X : Inport  Port=3
  Robot_Position_Y : Inport  Port=4
  Hypot : Math  Operator=hypot
  Subtract : Sum  Inputs=+-
  Subtract1 : Sum  Inputs=+-
  shot_distance : Outport
  wires:
  Hypot/1 -> shot_distance/1  "shot_distance"
  Subtract1/1 -> Hypot/2
  Subtract/1 -> Hypot/1
  Desired_Target_Y/1 -> Subtract1/1
  Robot_Position_Y/1 -> Subtract1/2
  Desired_Target_X/1 -> Subtract/1
  Robot_Position_X/1 -> Subtract/2

== system Shooting_Parameters_sub/Iterate_Shot_Target/Shot Distance to TOF ==
  shot_distance : Inport
  Shot_Distance_Lookup_Axis : Inport  Port=2
  Constant : Constant  Value=Rebuilt_Shoot_TOF_0
  Constant1 : Constant  Value=Rebuilt_Shoot_TOF_1
  Constant11 : Constant  Value=Rebuilt_Shoot_TOF_5
  Constant2 : Constant  Value=Rebuilt_Shoot_TOF_2
  Constant3 : Constant  Value=Rebuilt_Shoot_TOF_3
  Constant4 : Constant  Value=Rebuilt_Shoot_TOF_4
  Constant5 : Constant  Value=Rebuilt_Shoot_TOF_7
  Constant6 : Constant  Value=Rebuilt_Shoot_TOF_6
  Lookup Table Dynamic : simulink/Lookup Tables/Lookup Table Dynamic  LookUpMeth=Interpolation-Use End Values  OutDataType=fixdt('double')  OutScaling=[]  OutputDataTypeScalingMode=Specify via dialog  OutDataTypeStr=double  DoSatur=off
  Mux1 : Mux  Inputs=8
  TOF : Outport
  wires:
  Constant5/1 -> Mux1/8
  Constant6/1 -> Mux1/7
  Shot_Distance_Lookup_Axis/1 -> Lookup Table Dynamic/2
  Constant11/1 -> Mux1/6
  Lookup Table Dynamic/1 -> TOF/1  "TOF"
  Mux1/1 -> Lookup Table Dynamic/3  "TOF"
  shot_distance/1 -> Lookup Table Dynamic/1
  Constant1/1 -> Mux1/2
  Constant2/1 -> Mux1/3
  Constant3/1 -> Mux1/4
  Constant4/1 -> Mux1/5
  Constant/1 -> Mux1/1

== system Shooting_Parameters_sub/Iterate_Shot_Target/Target_Selection ==
  note: Target Selection
  note: This subsystem will feed in the input targets for the first loop, then feed in the previously-calculated targets for each successive loop.
  iteration_number : Inport
  Hub_X : Inport  Port=2
  Hub_Y : Inport  Port=3
  Desired_Target_X_Prev : Inport  Port=4
  Desired_Target_Y_Prev : Inport  Port=5
  Bus Creator : BusCreator  Inputs=5
  Bus Selector : BusSelector  OutputSignals=Desired_Target_X_Prev,Iteration_Number,RB_Shoot_Target_X
  Bus Selector1 : BusSelector  OutputSignals=Desired_Target_Y_Prev,Iteration_Number,RB_Shoot_Target_Y
  Switch : Switch  Criteria=u2 > Threshold  Threshold=1  SaturateOnIntegerOverflow=off  InputSameDT=off
  Switch1 : Switch  Criteria=u2 > Threshold  Threshold=1  SaturateOnIntegerOverflow=off  InputSameDT=off
  Desired_Target_X : Outport
  Desired_Target_Y : Outport  Port=2
  wires:
  Switch1/1 -> Desired_Target_Y/1  "Desired_Target_Y"
  Switch/1 -> Desired_Target_X/1  "Desired_Target_X"
  Bus Selector/3 -> Switch/3  "<RB_Shoot_Target_X>"
  Bus Selector/2 -> Switch/2  "<Iteration_Number>"
  Bus Selector/1 -> Switch/1  "<Desired_Target_X_Prev>"
  Bus Selector1/3 -> Switch1/3  "<RB_Shoot_Target_Y>"
  Bus Selector1/2 -> Switch1/2  "<Iteration_Number>"
  Bus Selector1/1 -> Switch1/1  "<Desired_Target_Y_Prev>"
  Bus Creator/1 -> Bus Selector/1, Bus Selector1/1
  Hub_X/1 -> Bus Creator/2
  Desired_Target_X_Prev/1 -> Bus Creator/4
  Hub_Y/1 -> Bus Creator/3
  iteration_number/1 -> Bus Creator/1
  Desired_Target_Y_Prev/1 -> Bus Creator/5

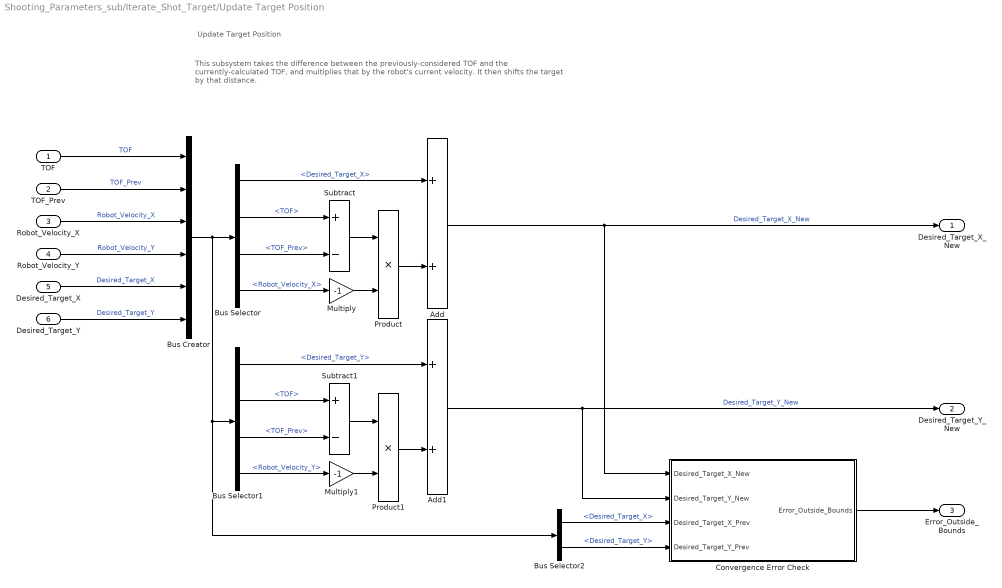
== system Shooting_Parameters_sub/Iterate_Shot_Target/Update Target Position ==
  note: Update Target Position
  note: This subsystem takes the difference between the previously-considered TOF and the currently-calculated TOF, and multiplies that by the robot's current velocity. It then shifts the target by that distance.
  TOF : Inport
  TOF_Prev : Inport  Port=2
  Robot_Velocity_X : Inport  Port=3
  Robot_Velocity_Y : Inport  Port=4
  Desired_Target_X : Inport  Port=5
  Desired_Target_Y : Inport  Port=6
  Add : Sum
  Add1 : Sum
  Bus Creator : BusCreator  Inputs=6
  Bus Selector : BusSelector  OutputSignals=Desired_Target_X,TOF,TOF_Prev,Robot_Velocity_X
  Bus Selector1 : BusSelector  OutputSignals=Desired_Target_Y,TOF,TOF_Prev,Robot_Velocity_Y
  Bus Selector2 : BusSelector  OutputSignals=Desired_Target_X,Desired_Target_Y
  Convergence Error Check : Subsystem
  Multiply : Gain  Gain=-1
  Multiply1 : Gain  Gain=-1
  Product : Product
  Product1 : Product
  Subtract : Sum  Inputs=+-
  Subtract1 : Sum  Inputs=+-
  Desired_Target_X_New : Outport
  Desired_Target_Y_New : Outport  Port=2
  Error_Outside_Bounds : Outport  Port=3
  wires:
  Bus Selector1/4 -> Multiply1/1  "<Robot_Velocity_Y>"
  Bus Selector1/3 -> Subtract1/2  "<TOF_Prev>"
  Bus Selector1/2 -> Subtract1/1  "<TOF>"
  Multiply1/1 -> Product1/2
  Subtract1/1 -> Product1/1
  Subtract/1 -> Product/1
  Bus Selector/2 -> Subtract/1  "<TOF>"
  Bus Selector/3 -> Subtract/2  "<TOF_Prev>"
  TOF_Prev/1 -> Bus Creator/2  "TOF_Prev"
  Bus Selector2/2 -> Convergence Error Check/4(Desired_Target_Y_Prev)  "<Desired_Target_Y>"
  Bus Selector2/1 -> Convergence Error Check/3(Desired_Target_X_Prev)  "<Desired_Target_X>"
  Convergence Error Check/1(Error_Outside_Bounds) -> Error_Outside_Bounds/1
  Add1/1 -> Convergence Error Check/2(Desired_Target_Y_New), Desired_Target_Y_New/1  "Desired_Target_Y_New"
  Bus Creator/1 -> Bus Selector/1, Bus Selector1/1, Bus Selector2/1
  Bus Selector1/1 -> Add1/1  "<Desired_Target_Y>"
  Product1/1 -> Add1/2
  Add/1 -> Desired_Target_X_New/1, Convergence Error Check/1(Desired_Target_X_New)  "Desired_Target_X_New"
  Product/1 -> Add/2
  Multiply/1 -> Product/2
  Bus Selector/4 -> Multiply/1  "<Robot_Velocity_X>"
  Bus Selector/1 -> Add/1  "<Desired_Target_X>"
  Desired_Target_X/1 -> Bus Creator/5  "Desired_Target_X"
  TOF/1 -> Bus Creator/1  "TOF"
  Desired_Target_Y/1 -> Bus Creator/6  "Desired_Target_Y"
  Robot_Velocity_X/1 -> Bus Creator/3  "Robot_Velocity_X"
  Robot_Velocity_Y/1 -> Bus Creator/4  "Robot_Velocity_Y"

== system Shooting_Parameters_sub/Look Up Desired Shooter Motor Speed/Rebuilt_Shoot_Shooter_Spd Init Array ==
  Constant1 : Constant  Value=Rebuilt_Shoot_Shooter_Spd_I_7
  Constant10 : Constant  Value=Rebuilt_Shoot_Shooter_Spd_I_5
  Constant2 : Constant  Value=Rebuilt_Shoot_Shooter_Spd_I_6
  Constant5 : Constant  Value=Rebuilt_Shoot_Shooter_Spd_I_0
  Constant6 : Constant  Value=Rebuilt_Shoot_Shooter_Spd_I_1
  Constant7 : Constant  Value=Rebuilt_Shoot_Shooter_Spd_I_2
  Constant8 : Constant  Value=Rebuilt_Shoot_Shooter_Spd_I_3
  Constant9 : Constant  Value=Rebuilt_Shoot_Shooter_Spd_I_4
  Mux : Mux  Inputs=8
  Rebuilt_Shoot_Shooter_Spd_I : Outport
  wires:
  Mux/1 -> Rebuilt_Shoot_Shooter_Spd_I/1
  Constant6/1 -> Mux/2
  Constant7/1 -> Mux/3
  Constant10/1 -> Mux/6
  Constant5/1 -> Mux/1
  Constant9/1 -> Mux/5
  Constant2/1 -> Mux/7
  Constant1/1 -> Mux/8
  Constant8/1 -> Mux/4

== system Shooting_Parameters_sub/Look Up Desired Shooter Motor Speed/Rebuilt_Shoot_Shooter_Spd Steady State Array ==
  Constant1 : Constant  Value=Rebuilt_Shoot_Shooter_Spd_7
  Constant10 : Constant  Value=Rebuilt_Shoot_Shooter_Spd_5
  Constant2 : Constant  Value=Rebuilt_Shoot_Shooter_Spd_6
  Constant5 : Constant  Value=Rebuilt_Shoot_Shooter_Spd_0
  Constant6 : Constant  Value=Rebuilt_Shoot_Shooter_Spd_1
  Constant7 : Constant  Value=Rebuilt_Shoot_Shooter_Spd_2
  Constant8 : Constant  Value=Rebuilt_Shoot_Shooter_Spd_3
  Constant9 : Constant  Value=Rebuilt_Shoot_Shooter_Spd_4
  Mux : Mux  Inputs=8
  Rebuilt_Shoot_Shooter_Spd : Outport
  wires:
  Mux/1 -> Rebuilt_Shoot_Shooter_Spd/1
  Constant6/1 -> Mux/2
  Constant7/1 -> Mux/3
  Constant10/1 -> Mux/6
  Constant5/1 -> Mux/1
  Constant9/1 -> Mux/5
  Constant2/1 -> Mux/7
  Constant1/1 -> Mux/8
  Constant8/1 -> Mux/4

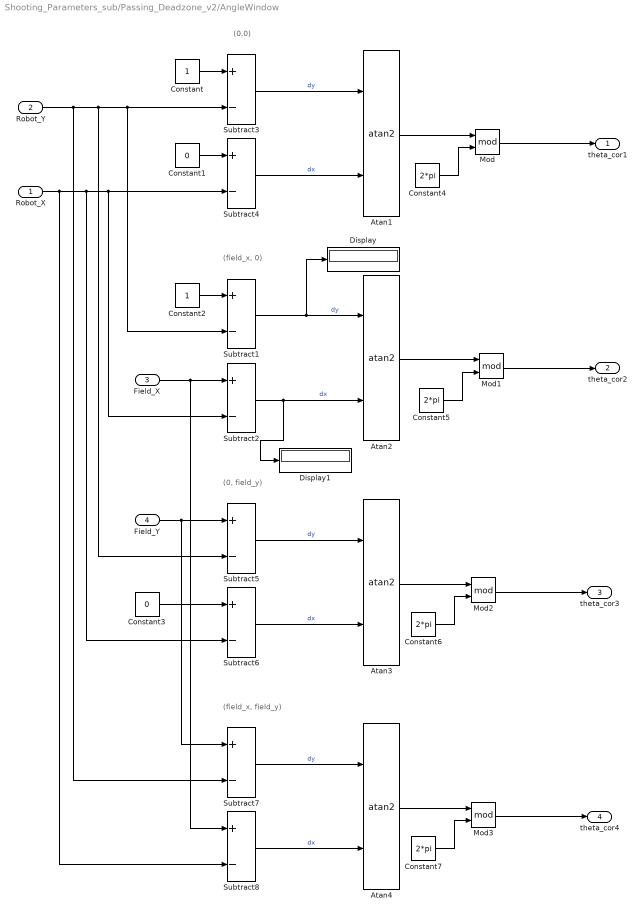
== system Shooting_Parameters_sub/Passing_Deadzone_v2/AngleWindow ==
  note: (field_x, field_y)
  note: (0, field_y)
  note: (field_x, 0)
  note: (0,0)
  Robot_X : Inport
  Robot_Y : Inport  Port=2
  Field_X : Inport  Port=3
  Field_Y : Inport  Port=4
  Atan{1..4} (4 alike) : Trigonometry  Operator=atan2
  Constant : Constant
  Constant1 : Constant  Value=0
  Constant2 : Constant
  Constant3 : Constant  Value=0
  Constant{4..7} (4 alike) : Constant  Value=2*pi
  Display : Display
  Display1 : Display
  Mod{,1..3} (4 alike) : Math  Operator=mod
  Subtract{1..8} (8 alike) : Sum  Inputs=+-
  theta_cor1 : Outport
  theta_cor2 : Outport  Port=2
  theta_cor3 : Outport  Port=3
  theta_cor4 : Outport  Port=4
  wires:
  Atan4/1 -> Mod3/1
  Constant7/1 -> Mod3/2
  Mod3/1 -> theta_cor4/1
  Atan3/1 -> Mod2/1
  Constant6/1 -> Mod2/2
  Mod2/1 -> theta_cor3/1
  Atan2/1 -> Mod1/1
  Constant5/1 -> Mod1/2
  Mod1/1 -> theta_cor2/1
  Mod/1 -> theta_cor1/1
  Constant4/1 -> Mod/2
  Atan1/1 -> Mod/1
  Constant3/1 -> Subtract6/1
  Field_Y/1 -> Subtract5/1, Subtract7/1
  Constant2/1 -> Subtract1/1
  Field_X/1 -> Subtract2/1, Subtract8/1
  Robot_X/1 -> Subtract4/2, Subtract2/2, Subtract6/2, Subtract8/2
  Robot_Y/1 -> Subtract5/2, Subtract3/2, Subtract1/2, Subtract7/2
  Constant1/1 -> Subtract4/1
  Constant/1 -> Subtract3/1
  Subtract8/1 -> Atan4/2  "dx"
  Subtract7/1 -> Atan4/1  "dy"
  Subtract6/1 -> Atan3/2  "dx"
  Subtract5/1 -> Atan3/1  "dy"
  Subtract2/1 -> Atan2/2, Display1/1  "dx"
  Subtract1/1 -> Atan2/1, Display/1  "dy"
  Subtract4/1 -> Atan1/2  "dx"
  Subtract3/1 -> Atan1/1  "dy"

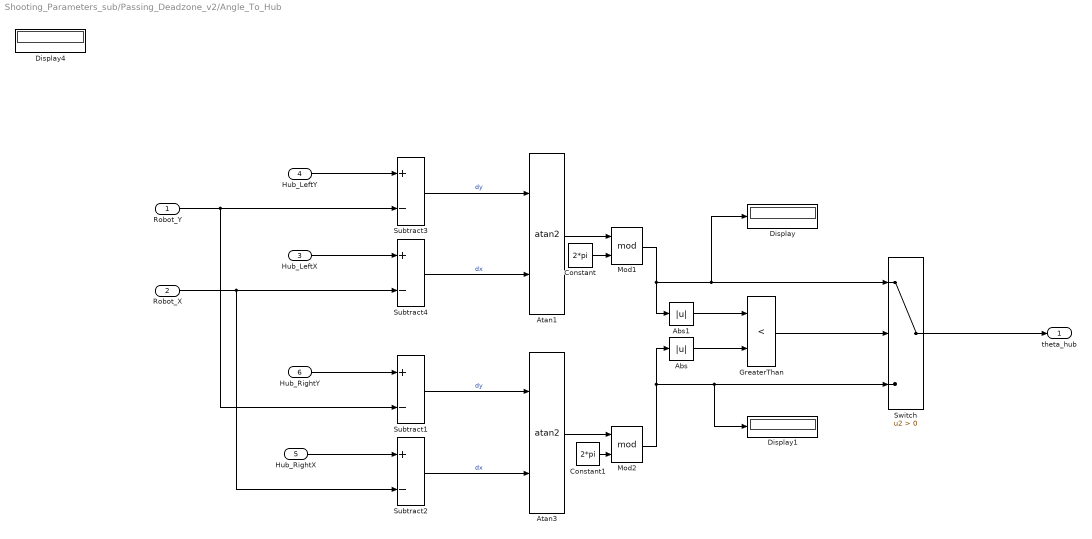
== system Shooting_Parameters_sub/Passing_Deadzone_v2/Angle_To_Hub ==
  Robot_Y : Inport
  Robot_X : Inport  Port=2
  Hub_LeftX : Inport  Port=3
  Hub_LeftY : Inport  Port=4
  Hub_RightX : Inport  Port=5
  Hub_RightY : Inport  Port=6
  Abs : Abs  SaturateOnIntegerOverflow=off
  Abs1 : Abs  SaturateOnIntegerOverflow=off
  Atan1 : Trigonometry  Operator=atan2
  Atan3 : Trigonometry  Operator=atan2
  Constant : Constant  Value=2*pi
  Constant1 : Constant  Value=2*pi
  Display : Display
  Display1 : Display
  Display4 : Display
  GreaterThan : RelationalOperator  Operator=<  OutDataTypeStr=boolean  RndMeth=Simplest  InputSameDT=off
  Mod1 : Math  Operator=mod  SignedPower=on
  Mod2 : Math  Operator=mod  SignedPower=on
  Subtract{1..4} (4 alike) : Sum  Inputs=+-
  Switch : Switch  Criteria=u2 > Threshold  SaturateOnIntegerOverflow=off  InputSameDT=off
  theta_hub : Outport
  wires:
  Atan3/1 -> Mod2/1
  Constant1/1 -> Mod2/2
  Subtract2/1 -> Atan3/2  "dx"
  Subtract1/1 -> Atan3/1  "dy"
  Mod2/1 -> Switch/3, Display1/1, Abs/1
  Mod1/1 -> Abs1/1, Switch/1, Display/1
  Constant/1 -> Mod1/2
  Atan1/1 -> Mod1/1
  Abs/1 -> GreaterThan/2
  Abs1/1 -> GreaterThan/1
  Switch/1 -> theta_hub/1
  GreaterThan/1 -> Switch/2
  Hub_RightY/1 -> Subtract1/1
  Hub_RightX/1 -> Subtract2/1
  Hub_LeftX/1 -> Subtract4/1
  Hub_LeftY/1 -> Subtract3/1
  Robot_X/1 -> Subtract2/2, Subtract4/2
  Robot_Y/1 -> Subtract1/2, Subtract3/2
  Subtract3/1 -> Atan1/1  "dy"
  Subtract4/1 -> Atan1/2  "dx"

== system Shooting_Parameters_sub/Passing_Deadzone_v2/Choose_Corner ==
  theta_cor1 : Inport
  theta_cor2 : Inport  Port=2
  theta_cor3 : Inport  Port=3
  theta_cor4 : Inport  Port=4
  Target_X : Inport  Port=5
  Target_Y : Inport  Port=6
  If : If  IfExpression=u1 > Field_Hub_Y
  If Action Subsystem : Subsystem  TreatAsAtomicUnit=on
  If Action Subsystem1 : Subsystem  TreatAsAtomicUnit=on
  Merge : Merge
  theta_corner : Outport
  wires:
  theta_cor4/1 -> If Action Subsystem/2(theta_cor4)
  theta_cor3/1 -> If Action Subsystem/1(theta_cor3)
  theta_cor2/1 -> If Action Subsystem1/2(theta_cor2)
  Target_X/1 -> If Action Subsystem/3(Target_X), If Action Subsystem1/3(Target_X)
  Merge/1 -> theta_corner/1
  If Action Subsystem1/1(theta_corner) -> Merge/2
  If Action Subsystem/1(theta_corner) -> Merge/1
  theta_cor1/1 -> If Action Subsystem1/1(theta_cor1)
  If/2 -> If Action Subsystem1/Action
  Target_Y/1 -> If/1
  If/1 -> If Action Subsystem/Action

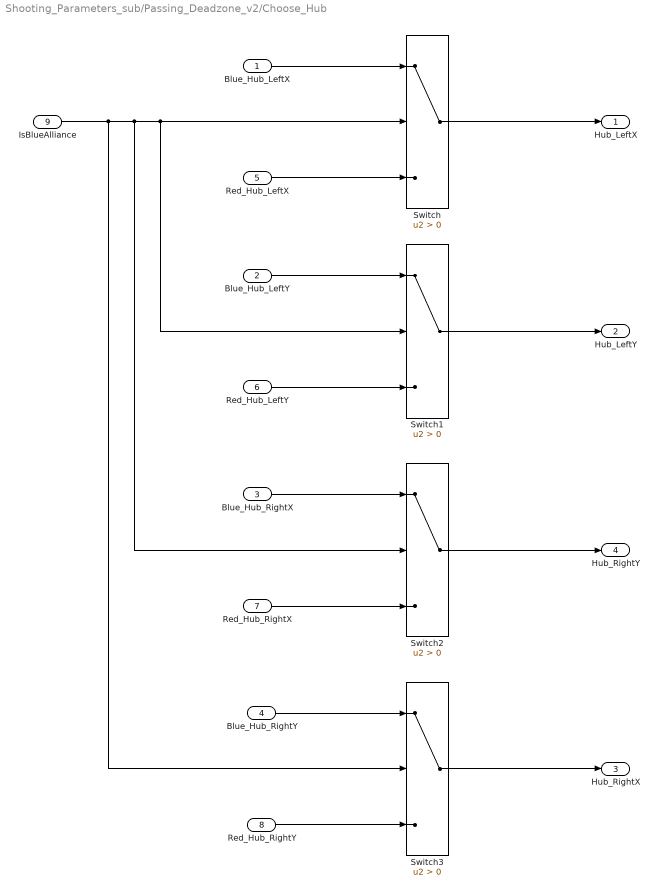
== system Shooting_Parameters_sub/Passing_Deadzone_v2/Choose_Hub ==
  Blue_Hub_LeftX : Inport
  Blue_Hub_LeftY : Inport  Port=2
  Blue_Hub_RightX : Inport  Port=3
  Blue_Hub_RightY : Inport  Port=4
  Red_Hub_LeftX : Inport  Port=5
  Red_Hub_LeftY : Inport  Port=6
  Red_Hub_RightX : Inport  Port=7
  Red_Hub_RightY : Inport  Port=8
  IsBlueAlliance : Inport  Port=9
  Switch{,1..3} (4 alike) : Switch  Criteria=u2 > Threshold  SaturateOnIntegerOverflow=off  InputSameDT=off
  Hub_LeftX : Outport
  Hub_LeftY : Outport  Port=2
  Hub_RightX : Outport  Port=3
  Hub_RightY : Outport  Port=4
  wires:
  Red_Hub_LeftX/1 -> Switch/3
  Blue_Hub_RightY/1 -> Switch3/1
  Red_Hub_RightY/1 -> Switch3/3
  Red_Hub_RightX/1 -> Switch2/3
  Blue_Hub_RightX/1 -> Switch2/1
  Blue_Hub_LeftY/1 -> Switch1/1
  Red_Hub_LeftY/1 -> Switch1/3
  Blue_Hub_LeftX/1 -> Switch/1
  Switch3/1 -> Hub_RightX/1
  Switch2/1 -> Hub_RightY/1
  Switch1/1 -> Hub_LeftY/1
  Switch/1 -> Hub_LeftX/1
  IsBlueAlliance/1 -> Switch3/2, Switch2/2, Switch1/2, Switch/2

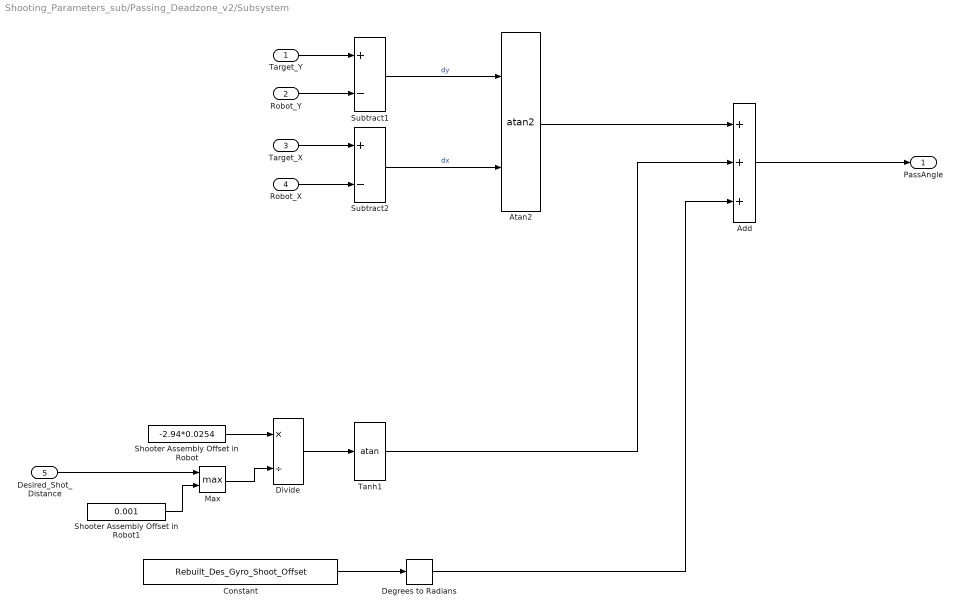
== system Shooting_Parameters_sub/Passing_Deadzone_v2/Subsystem ==
  Target_Y : Inport
  Robot_Y : Inport  Port=2
  Target_X : Inport  Port=3
  Robot_X : Inport  Port=4
  Desired_Shot_Distance : Inport  Port=5
  Add : Sum  Inputs=+++
  Atan2 : Trigonometry  Operator=atan2
  Constant : Constant  Value=Rebuilt_Des_Gyro_Shoot_Offset
  Degrees to Radians : simulink_extras/Transformations/Degrees to Radians
  Divide : Product  Inputs=*/
  Max : MinMax  Function=max  Inputs=2
  Shooter Assembly Offset in Robot : Constant  Value=-2.94*0.0254
  Shooter Assembly Offset in Robot1 : Constant  Value=0.001
  Subtract1 : Sum  Inputs=+-
  Subtract2 : Sum  Inputs=+-
  Tanh1 : Trigonometry  Operator=atan
  PassAngle : Outport
  wires:
  Degrees to Radians/1 -> Add/3
  Atan2/1 -> Add/1
  Add/1 -> PassAngle/1
  Constant/1 -> Degrees to Radians/1
  Tanh1/1 -> Add/2
  Desired_Shot_Distance/1 -> Max/1
  Divide/1 -> Tanh1/1
  Shooter Assembly Offset in Robot1/1 -> Max/2
  Shooter Assembly Offset in Robot/1 -> Divide/1
  Max/1 -> Divide/2
  Robot_Y/1 -> Subtract1/2
  Robot_X/1 -> Subtract2/2
  Target_Y/1 -> Subtract1/1
  Subtract1/1 -> Atan2/1  "dy"
  Subtract2/1 -> Atan2/2  "dx"
  Target_X/1 -> Subtract2/1

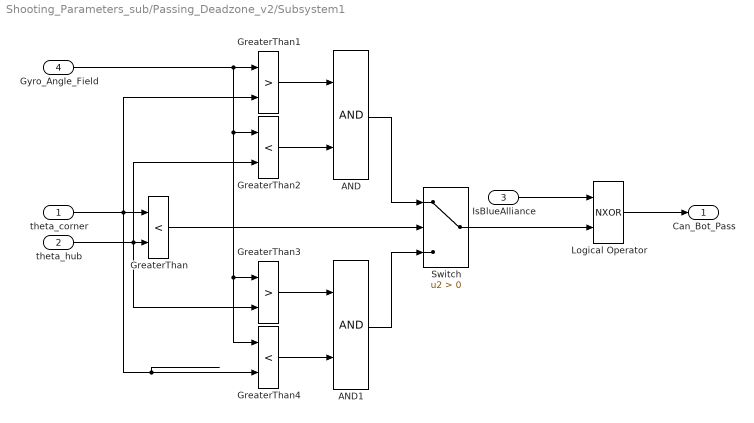
== system Shooting_Parameters_sub/Passing_Deadzone_v2/Subsystem1 ==
  theta_corner : Inport
  theta_hub : Inport  Port=2
  IsBlueAlliance : Inport  Port=3
  Gyro_Angle_Field : Inport  Port=4
  AND : Logic  AllPortsSameDT=off  OutDataTypeStr=boolean
  AND1 : Logic  AllPortsSameDT=off  OutDataTypeStr=boolean
  GreaterThan : RelationalOperator  Operator=<  OutDataTypeStr=boolean  RndMeth=Simplest  InputSameDT=off
  GreaterThan1 : RelationalOperator  Operator=>  OutDataTypeStr=boolean  RndMeth=Simplest  InputSameDT=off
  GreaterThan2 : RelationalOperator  Operator=<  OutDataTypeStr=boolean  RndMeth=Simplest  InputSameDT=off
  GreaterThan3 : RelationalOperator  Operator=>  OutDataTypeStr=boolean  RndMeth=Simplest  InputSameDT=off
  GreaterThan4 : RelationalOperator  Operator=<  OutDataTypeStr=boolean  RndMeth=Simplest  InputSameDT=off
  Logical Operator : Logic  Operator=NXOR  AllPortsSameDT=off  OutDataTypeStr=boolean
  Switch : Switch  Criteria=u2 > Threshold  SaturateOnIntegerOverflow=off  InputSameDT=off
  Can_Bot_Pass : Outport
  wires:
  AND1/1 -> Switch/3
  IsBlueAlliance/1 -> Logical Operator/1
  Logical Operator/1 -> Can_Bot_Pass/1
  Switch/1 -> Logical Operator/2
  GreaterThan/1 -> Switch/2
  AND/1 -> Switch/1
  GreaterThan4/1 -> AND1/2
  GreaterThan3/1 -> AND1/1
  GreaterThan2/1 -> AND/2
  GreaterThan1/1 -> AND/1
  Gyro_Angle_Field/1 -> GreaterThan1/1, GreaterThan2/1, GreaterThan3/1, GreaterThan4/1
  theta_hub/1 -> GreaterThan/2, GreaterThan3/2, GreaterThan2/2
  theta_corner/1 -> GreaterThan/1, GreaterThan4/2, GreaterThan1/2

== system Shooting_Parameters_sub/Iterate_Shot_Target/Update Target Position/Convergence Error Check ==
  note: Convergence Error Check
  note: Another simple distance check, this will allow us to stop iterating if we're "close enough"
  Desired_Target_X_New : Inport
  Desired_Target_Y_New : Inport  Port=2
  Desired_Target_X_Prev : Inport  Port=3
  Desired_Target_Y_Prev : Inport  Port=4
  Compare To Constant : simulink/Logic and Bit Operations/Compare To Constant  relop=>=  const=Rebuilt_Shoot_Target_Error_Thresh  OutDataTypeStr=boolean
  Hypot : Math  Operator=hypot
  Subtract : Sum  Inputs=+-
  Subtract1 : Sum  Inputs=+-
  Error_Outside_Bounds : Outport
  wires:
  Compare To Constant/1 -> Error_Outside_Bounds/1  "Error_Outside_Bounds"
  Hypot/1 -> Compare To Constant/1
  Desired_Target_Y_Prev/1 -> Subtract1/2  "Desired_Target_Y_Prev"
  Desired_Target_Y_New/1 -> Subtract1/1  "Desired_Target_Y"
  Desired_Target_X_New/1 -> Subtract/1  "Desired_Target_X"
  Desired_Target_X_Prev/1 -> Subtract/2  "Desired_Target_X_Prev"
  Subtract/1 -> Hypot/1
  Subtract1/1 -> Hypot/2

== system Shooting_Parameters_sub/Passing_Deadzone_v2/Choose_Corner/If Action Subsystem ==
  theta_cor3 : Inport
  theta_cor4 : Inport  Port=2
  Target_X : Inport  Port=3
  Action Port : ActionPort
  Switch : Switch  Criteria=u2 > Threshold  Threshold=Field_Length_Half  SaturateOnIntegerOverflow=off  InputSameDT=off
  theta_corner : Outport
  wires:
  Switch/1 -> theta_corner/1
  theta_cor3/1 -> Switch/3
  theta_cor4/1 -> Switch/1
  Target_X/1 -> Switch/2

== system Shooting_Parameters_sub/Passing_Deadzone_v2/Choose_Corner/If Action Subsystem1 ==
  theta_cor1 : Inport
  theta_cor2 : Inport  Port=2
  Target_X : Inport  Port=3
  Action Port : ActionPort
  Switch : Switch  Criteria=u2 > Threshold  Threshold=Field_Length_Half  SaturateOnIntegerOverflow=off  InputSameDT=off
  theta_corner : Outport
  wires:
  Switch/1 -> theta_corner/1
  theta_cor1/1 -> Switch/3
  theta_cor2/1 -> Switch/1
  Target_X/1 -> Switch/2
